simulink model "slex2"  (R2018b)
settings: Solver=FixedStepAuto  StartTime=0.0  StopTime=10.0  FixedStep=0.01  RelTol=1e-3
settings Model: Creator=19810  LastModifiedBy=19810
settings DataIOCC: InspectSignalLogs=on

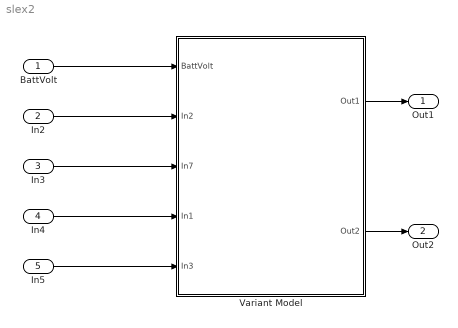
== system slex2 ==
  BattVolt : Inport
  In2 : Inport  Port=2
  In3 : Inport  Port=3
  In4 : Inport  Port=4
  In5 : Inport  Port=5
  Variant Model : Subsystem  Variant=on
  Out1 : Outport
  Out2 : Outport  Port=2
  wires:
  BattVolt/1 -> Variant Model/1("BattVolt ")
  In2/1 -> Variant Model/2(In2)
  In3/1 -> Variant Model/3(In7)
  In4/1 -> Variant Model/4(In1)
  Variant Model/1(Out1) -> Out1/1
  In5/1 -> Variant Model/5(In3)
  Variant Model/2(Out2) -> Out2/1

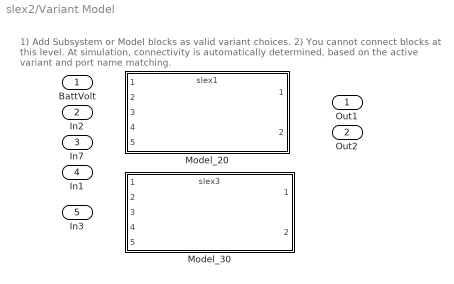
== system slex2/Variant Model ==
  note: 1) Add Subsystem or Model blocks as valid variant choices.
      | 2) You cannot connect blocks at this level. At simulation, connectivity is automatically
      | determined, based on the active variant and port name matching.
  "BattVolt " : Inport
  In2 : Inport  Port=2
  In7 : Inport  Port=3
  In1 : Inport  Port=4
  In3 : Inport  Port=5
  Model_20 : ModelReference  DisableCoverage=on  ModelNameDialog=slex1.slx  VariantControl=k == 1  ModelReferenceVersion=1.15
  Model_30 : ModelReference  ModelNameDialog=slex3.slx  VariantControl=k == 2  ModelReferenceVersion=1.8
  Out1 : Outport
  Out2 : Outport  Port=2
